simulink model "Problem1"  (R2026a)
settings: Solver=VariableStepAuto
model workspace (MAT data in the model file):
  X = 1
undefined symbols (not defined in the file or in its folder): i
libraries: dspinverses x1
settings Model: Creator=rawad  LastModifiedBy=rawad

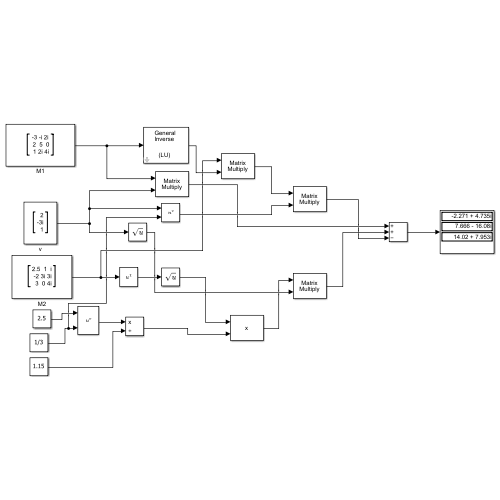
[thumbnail: Simulink's stored preview of the top-level diagram]
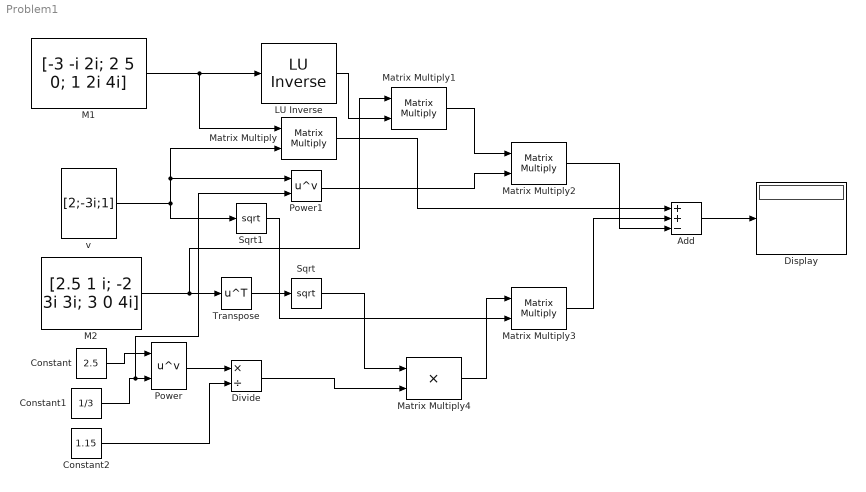
== system Problem1 ==
  " LU Inverse" : dspinverses/ LU Inverse
  Add : Sum  Inputs=++-
  Constant : Constant  Value=2.5
  Constant1 : Constant  Value=1/3
  Constant2 : Constant  Value=1.15
  Display : Display
  Divide : Product  Inputs=*/
  M1 : Constant  Value=[-3 -i 2i; 2 5 0; 1 2i 4i]  VectorParams1D=off
  M2 : Constant  Value=[2.5 1 i; -2 3i 3i; 3 0 4i]  VectorParams1D=off
  Matrix Multiply{,1..3} (4 alike) : Product  Multiplication=Matrix(*)
  Matrix Multiply4 : Product
  Power : Math  Operator=pow
  Power1 : Math  Operator=pow
  Sqrt : Sqrt
  Sqrt1 : Sqrt
  Transpose : Math  Operator=transpose
  v : Constant  Value=[2;-3i;1]  VectorParams1D=off
  wires:
  M1/1 -> " LU Inverse"/1, Matrix Multiply/1
  v/1 -> Sqrt1/1, Matrix Multiply/2, Power1/1
  M2/1 -> Matrix Multiply1/1, Transpose/1
  Transpose/1 -> Sqrt/1
  Constant/1 -> Power/1
  Constant1/1 -> Power1/2, Power/2
  Power/1 -> Divide/1
  Constant2/1 -> Divide/2
  Matrix Multiply1/1 -> Matrix Multiply2/1
  Power1/1 -> Matrix Multiply2/2
  Sqrt/1 -> Matrix Multiply4/1
  Sqrt1/1 -> Matrix Multiply3/2
  Matrix Multiply/1 -> Add/1
  Matrix Multiply2/1 -> Add/3
  Add/1 -> Display/1
  Divide/1 -> Matrix Multiply4/2
  Matrix Multiply4/1 -> Matrix Multiply3/1
  Matrix Multiply3/1 -> Add/2
  " LU Inverse"/1 -> Matrix Multiply1/2
